simulink model "SpaceKinova_Torque"  (R2025b)
settings: Solver=ode14x  StartTime=0.0  StopTime=8.5  FixedStep=0.005  RelTol=1e-3
undefined symbols (not defined in the file): d_safe, dspblkCoreblockFVToolHelper, gcbh, isdone_init, reward_init, X, Y, Z
libraries: sm_lib x98, nesl_utility x50, rllib x1, sharedutil x1
(part 3 of 3)

== matlab function SpaceKinova_Torque/collision monitor/MATLAB Function ==
  data: q input; dmin output; isColl output
function [dmin,isColl] = collisionMonitorFcn(q)
    %#codegen
    
    coder.extrinsic('collisionCheckWrapper');
    
    % feste Outputs initialisieren
    dmin   = inf;
    isColl = false;
    
    % q auf 1x4 bringen (keine dynamische Größe!)
    nJ   = 4;
    qrow = zeros(1,nJ);
    
    L = min(numel(q), nJ);
    q_flat = reshape(q(1:L),1,[]);
    qrow(1,1:L) = q_flat;
    
    % extrinsische Kollisionsfunktion aufrufen
    dmin_ext   = dmin;
    isColl_ext = isColl;
    
    [dmin_ext, isColl_ext] = collisionCheckWrapper(qrow);
    
    dmin   = dmin_ext;
    isColl = isColl_ext;

end

== matlab function SpaceKinova_Torque/Reward/MATLAB Function ==
  data: ep input; reward output; ev input; dq_cmd input; dq_cmd_prev input; isDone output
function [reward, isDone] = rewardFcn(ep, ev, dq_cmd, dq_cmd_prev)

    if any(~isfinite([ep; ev; dq_cmd; dq_cmd_prev]))
        reward = -50;
        isDone = true;
        return;
    end

    dist = norm(ep);
    vel  = norm(ev);

    if dist > 0.5 || vel > 2
        reward = -50;
        isDone = true;
        return;
    end

    c_pos = min(ep.' * ep, 0.25);      % clip
    c_vel = min(ev.' * ev, 4.0);       % clip
    c_u   = min(dq_cmd.' * dq_cmd, 10);
    c_du  = min((dq_cmd-dq_cmd_prev).' * (dq_cmd-dq_cmd_prev), 10);

    reward = ...
        - 20 * c_pos ...
        -  2 * c_vel ...
        -  0.02 * c_u ...
        -  0.05 * c_du;

    if dist < 0.05
        reward = reward + 1;
    end

    if dist < 0.02
        reward = reward + 3;
    end

    isDone = false;
end

== matlab function SpaceKinova_Torque/Robot/Impuls Monitor/MATLAB Function ==
  data: v1 input; p_tot output; w1 input; q1 input; v2 input; w2 input; q2 input; v3 input; w3 input; q3 input; v4 input; w4 input; q4 input; v5 input; w5 input; q5 input
function p_tot = totalMomentum( ...
    v1,w1,q1, ...
    v2,w2,q2, ...
    v3,w3,q3, ...
    v4,w4,q4, ...
    v5,w5,q5)

%#codegen

    % Massen
    m = [5; 1; 1; 1; 1];

    % COM-Offsets im jeweiligen Link-Frame
    r_link = [ 0.0  0.0  0.0;   % Link 1
               0.5  0.0  0.0;   % Link 2
               0.5  0.0  0.0;   % Link 3
               0.5  0.0  0.0;   % Link 4
               0.5  0.0  0.0];  % Link 5

    % Initialisiere Gesamtimpuls
    p_tot = zeros(3,1);

    % Link 1
    p_tot = p_tot + linkMomentum(v1, w1, q1, m(1), r_link(1,:).');

    % Link 2
    p_tot = p_tot + linkMomentum(v2, w2, q2, m(2), r_link(2,:).');

    % Link 3
    p_tot = p_tot + linkMomentum(v3, w3, q3, m(3), r_link(3,:).');

    % Link 4
    p_tot = p_tot + linkMomentum(v4, w4, q4, m(4), r_link(4,:).');

    % Link 5
    p_tot = p_tot + linkMomentum(v5, w5, q5, m(5), r_link(5,:).');

end

function p = linkMomentum(v, w, q, m, r_link)
% v, w: 3x1 im World-Frame
% q: 4x1 Quaternion [w x y z], Orientierung Link relativ zu World
% r_link: 3x1 COM-Offset im Link-Frame

    % COM-Offset in World-Koordinaten drehen
    r_world = quatRotate(q, r_link);

    % COM-Geschwindigkeit
    v_com = v + cross(w, r_world);

    % Impuls dieses Links
    p = m * v_com;
end

function v_out = quatRotate(q, v_in)
% rotiert v_in (3x1) mit Quaternion q = [w x y z]

    % Normalisieren zur Sicherheit
    q = q(:) / norm(q);

    w = q(1);
    x = q(2);
    y = q(3);
    z = q(4);

    % Rotationsmatrix aus Quaternion (world <- link)
    R = [1-2*(y^2+z^2),   2*(x*y - z*w),   2*(x*z + y*w);
         2*(x*y + z*w),   1-2*(x^2+z^2),   2*(y*z - x*w);
         2*(x*z - y*w),   2*(y*z + x*w),   1-2*(x^2+y^2)];

    v_out = R * v_in(:);
end

== matlab function SpaceKinova_Torque/Robot/MATLAB Function2 ==
  data: q0 input; e_ori output; qb input
function e_ori = quatOriError(q0, qb)

    if qb(1) < 0, qb = -qb; end
    
    % ensure unit quaternions
    q0 = q0(:)/norm(q0); qb = qb(:)/norm(qb);
    
    % relative: q_err = conj(q0) * qb
    qconj = [ q0(1); -q0(2:4) ];
    qerr  = quatMultiply(qconj, qb);
    
    % keep scalar part non-negative to avoid flips
    if qerr(1) < 0
        qerr = -qerr;
    end
    
    w = qerr(1);
    v = qerr(2:4);
    nv = norm(v);
    
    if nv < 1e-12
        e_ori = [0;0;0];
    else
        theta = 2*atan2(nv, max(1e-12, w));
        u = v / nv;
        e_ori = theta * u;   % 3x1
    end
end

function q = quatMultiply(q1,q2)
    % [w x y z] * [w x y z]
    w1=q1(1); v1=q1(2:4); w2=q2(1); v2=q2(2:4);
    w  = w1*w2 - dot(v1,v2);
    v  = w1*v2 + w2*v1 + cross(v1,v2);
    q  = [w; v];
end
